simulink library "cylPackParChnlsLumped"  (R2025a)
settings: Solver=VariableStepAuto  StartTime=0.0  StopTime=10.0  RelTol=1e-3
undefined symbols (not defined in the file or in its folder): battery_builder_rtmsupport, gcbh
libraries: cylPackParChnlsLumped_lib x10, nesl_utility x3, batt_lib x1
(part 1 of 2)
settings Model: Creator=SimuVerity Contributors  LastModifiedBy=SimuVerity Contributors

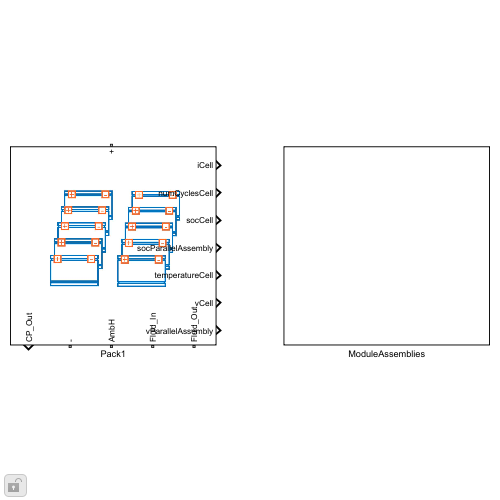
[thumbnail: Simulink's stored preview of the top-level diagram]
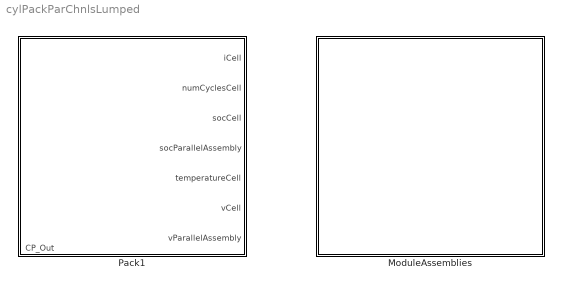
== system cylPackParChnlsLumped ==
  ModuleAssemblies : Subsystem
  Pack1 : Subsystem  LoadFcn=battery_builder_rtmsupport('loadfcn',gcbh);
      settings: CopyFcn=battery_builder_rtmsupport('copyfcn',gcbh);  PreCopyFcn=battery_builder_rtmsupport('precopyfcn',gcbh);  PreDeleteFcn=battery_builder_rtmsupport('predeletefcn',gcbh);  PortSchema="{\"entries\":[{\"content\":{\"sides\":[{\"content\":{\"connectorIds\":[\"LConn1\"]},\"type\":\"ConnectorPlacement.EquallySpacedRectSide\",\"uuid\":\"4681bb03-cd80-4246-89ba-52cf50faf921\"},{\"content\":{\"connectorIds\":[\"Out1\",\"RConn1\",\"RConn2\",\"RConn3\",\"RConn4\"],\"side\":\"RIGHT\"},\"type\":\"ConnectorPlacement.EquallySpacedRectSide\",\"uuid\":\"284cb137-d0f2-4bd0-b852-eba4066dd0c4\"},{\"content\":{\"side\":\"TOP\"},\"type\":\"ConnectorPlacement.EquallySpacedRectSide\",\"uuid\":\"dd50f81c-cf45-4e78-b3f5-c98c381b47a3\"},{\"content\":{\"connectorIds\":[\"Out2\",\"Out3\",\"Out4\",\"Out5\",\"Out6\",\"Out7\",\"Out8\"],\"side\":\"BOTTOM\"},\"type\":\"ConnectorPlacement.EquallySpacedRectSide\",\"uuid\":\"d30ee6a7-df81-42fc-8647-81cdeceb78f0\"}]},\"type\":\"ConnectorPlacement.EquallySpacedConnector\",\"uuid\":\"ee24a402-9efb-4b9e-88eb-dd7a5584ec7d\"}],\"packageUris\":[\"http://schema.mathworks.com/mf0/Connector/R2020b\"],\"version\":\"1.0\"}"
      mask Display: image('$imagefile')

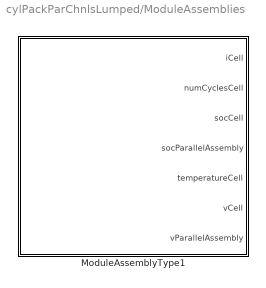
== system cylPackParChnlsLumped/ModuleAssemblies ==
  ModuleAssemblyType1 : Subsystem  LoadFcn=battery_builder_rtmsupport('loadfcn',gcbh);
      settings: CopyFcn=battery_builder_rtmsupport('copyfcn',gcbh);  PreCopyFcn=battery_builder_rtmsupport('precopyfcn',gcbh);  PreDeleteFcn=battery_builder_rtmsupport('predeletefcn',gcbh);  PortSchema="{\"entries\":[{\"content\":{\"sides\":[{\"content\":{\"connectorIds\":[\"LConn1\"]},\"type\":\"ConnectorPlacement.EquallySpacedRectSide\",\"uuid\":\"9f5d6674-91e5-41ab-bf84-a47b2d600243\"},{\"content\":{\"connectorIds\":[\"RConn1\",\"RConn2\",\"RConn3\"],\"side\":\"RIGHT\"},\"type\":\"ConnectorPlacement.EquallySpacedRectSide\",\"uuid\":\"fcae5f38-dd9a-4f90-b910-c15464afb2bd\"},{\"content\":{\"side\":\"TOP\"},\"type\":\"ConnectorPlacement.EquallySpacedRectSide\",\"uuid\":\"4b5634d1-8304-4a4e-97d4-9f8ecfb1b379\"},{\"content\":{\"connectorIds\":[\"Out1\",\"Out2\",\"Out3\",\"Out4\",\"Out5\",\"Out6\",\"Out7\"],\"side\":\"BOTTOM\"},\"type\":\"ConnectorPlacement.EquallySpacedRectSide\",\"uuid\":\"9ef905cb-dcbb-447b-9a1a-de2399b1e889\"}]},\"type\":\"ConnectorPlacement.EquallySpacedConnector\",\"uuid\":\"4a8d5c07-7366-4205-9241-e1a572108c18\"}],\"packageUris\":[\"http://schema.mathworks.com/mf0/Connector/R2020b\"],\"version\":\"1.0\"}"
      mask Display: image('$imagefile')

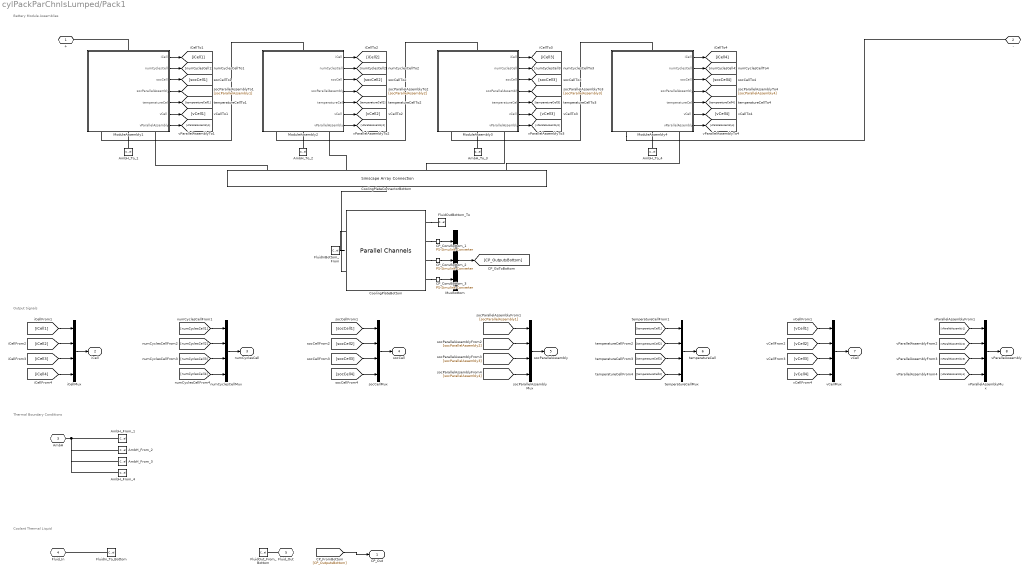
== system cylPackParChnlsLumped/Pack1 ==
  note: Battery Module Assemblies
  note: Output Signals
  note: Thermal Boundary Conditions
  note: Coolant Thermal Liquid
  AmbH_From_1 : ConnectionLabel  Label=ambH_1
  AmbH_From_2 : ConnectionLabel  Label=ambH_2
  AmbH_From_3 : ConnectionLabel  Label=ambH_3
  AmbH_From_4 : ConnectionLabel  Label=ambH_4
  AmbH_To_1 : ConnectionLabel  Label=ambH_1
  AmbH_To_2 : ConnectionLabel  Label=ambH_2
  AmbH_To_3 : ConnectionLabel  Label=ambH_3
  AmbH_To_4 : ConnectionLabel  Label=ambH_4
  CP_ConvBottom_1 : nesl_utility/PS-Simulink Converter  PhysicalDomain=network_engine_domain  SubClassName=ps_output  LeftPortType=input  RightPortType=output  PseudoPeriodic=off  Frequencies=[]  VectorFormat=inherit  Unit=inherit  AffineConversion=off
  CP_ConvBottom_2 : nesl_utility/PS-Simulink Converter  PhysicalDomain=network_engine_domain  SubClassName=ps_output  LeftPortType=input  RightPortType=output  PseudoPeriodic=off  Frequencies=[]  VectorFormat=inherit  Unit=inherit  AffineConversion=off
  CP_ConvBottom_3 : nesl_utility/PS-Simulink Converter  PhysicalDomain=network_engine_domain  SubClassName=ps_output  LeftPortType=input  RightPortType=output  PseudoPeriodic=off  Frequencies=[]  VectorFormat=inherit  Unit=inherit  AffineConversion=off
  CoolingPlateBottom : batt_lib/Thermal/Parallel Channels  plateConnectivity=simscape.battery.enum.thermal.coolingPlateConnectivity.singleSided  numBattThermalNodes1=CoolingPlateBottom.numBattThermalNodes1  dimensionThermalNodes1=CoolingPlateBottom.dimensionThermalNodes1  locationThermalNodes1=CoolingPlateBottom.locationThermalNodes1  numBattThermalNodes2=1  dimensionThermalNodes2=ones(1, 2)  locationThermalNodes2=ones(1, 2)  plateDimX=CoolingPlateBottom.plateDimX  plateDimY=CoolingPlateBottom.plateDimY  plateTh=CoolingPlateBottom.plateTh m  plateThCond=CoolingPlateBottom.plateThCond W/(K*m)  plateDen=CoolingPlateBottom.plateDen kg/m^3  plateCp=CoolingPlateBottom.plateCp J/(K*kg)  plateTemp_ini=CoolingPlateBottom.plateTemp_ini K  Re_lam=CoolingPlateBottom.Re_lam  Re_tur=CoolingPlateBottom.Re_tur  Nu_lam=CoolingPlateBottom.Nu_lam  length_add=CoolingPlateBottom.length_add m  shape_factor=CoolingPlateBottom.shape_factor  nChannels=CoolingPlateBottom.nChannels  selectChannelOrientation=simscape.battery.enum.thermal.coolingChannelsDirection.alongX  channelDia=CoolingPlateBottom.channelDia m  distributorDia=CoolingPlateBottom.distributorDia m  roughnessPipe=CoolingPlateBottom.roughnessPipe m
      settings: InternalSimscapePortConfiguration="{\"Bottom\":[],\"Left\":[{\"id\":\"fluid_in\",\"label\":\"fluid_in\",\"type\":\"foundation.thermal_liquid.thermal_liquid\"}],\"Right\":[{\"id\":\"fluid_out\",\"label\":\"fluid_out\",\"type\":\"foundation.thermal_liquid.thermal_liquid\"},{\"id\":\"plotPlateT\",\"label\":\"Tp\",\"type\":\"output\"},{\"id\":\"tempSensor\",\"label\":\"dT\",\"type\":\"output\"},{\"id\":\"presSensor\",\"label\":\"dP\",\"type\":\"output\"}],\"Top\":[{\"id\":\"Side1\",\"label\":\"Surf1\",\"type\":\"foundation.thermal.thermal\"}]}"
  CoolingPlateConnectorBottom : SimscapeArrayConnection  Domain=foundation.thermal.thermal  Mode=Sized Elements
  FluidInBottom_From : ConnectionLabel  Label=FluidIn_To_Bottom
  FluidIn_To_Bottom : ConnectionLabel  Label=FluidIn_To_Bottom
  FluidOutBottom_To : ConnectionLabel  Label=FluidOut_From_Bottom
  FluidOut_From_Bottom : ConnectionLabel  Label=FluidOut_From_Bottom
  ModuleAssembly1 : Subsystem  LoadFcn=battery_builder_rtmsupport('loadfcn',gcbh);
      settings: CopyFcn=battery_builder_rtmsupport('copyfcn',gcbh);  PreCopyFcn=battery_builder_rtmsupport('precopyfcn',gcbh);  PreDeleteFcn=battery_builder_rtmsupport('predeletefcn',gcbh);  PortSchema="{\"entries\":[{\"content\":{\"sides\":[{\"content\":{\"connectorIds\":[\"LConn1\"]},\"type\":\"ConnectorPlacement.EquallySpacedRectSide\",\"uuid\":\"9f5d6674-91e5-41ab-bf84-a47b2d600243\"},{\"content\":{\"connectorIds\":[\"RConn1\",\"RConn2\",\"RConn3\"],\"side\":\"RIGHT\"},\"type\":\"ConnectorPlacement.EquallySpacedRectSide\",\"uuid\":\"fcae5f38-dd9a-4f90-b910-c15464afb2bd\"},{\"content\":{\"side\":\"TOP\"},\"type\":\"ConnectorPlacement.EquallySpacedRectSide\",\"uuid\":\"4b5634d1-8304-4a4e-97d4-9f8ecfb1b379\"},{\"content\":{\"connectorIds\":[\"Out1\",\"Out2\",\"Out3\",\"Out4\",\"Out5\",\"Out6\",\"Out7\"],\"side\":\"BOTTOM\"},\"type\":\"ConnectorPlacement.EquallySpacedRectSide\",\"uuid\":\"9ef905cb-dcbb-447b-9a1a-de2399b1e889\"}]},\"type\":\"ConnectorPlacement.EquallySpacedConnector\",\"uuid\":\"4a8d5c07-7366-4205-9241-e1a572108c18\"}],\"packageUris\":[\"http://schema.mathworks.com/mf0/Connector/R2020b\"],\"version\":\"1.0\"}"
      mask Display: image('$imagefile')
  ModuleAssembly2 : Subsystem  LoadFcn=battery_builder_rtmsupport('loadfcn',gcbh);
      settings: CopyFcn=battery_builder_rtmsupport('copyfcn',gcbh);  PreCopyFcn=battery_builder_rtmsupport('precopyfcn',gcbh);  PreDeleteFcn=battery_builder_rtmsupport('predeletefcn',gcbh);  PortSchema="{\"entries\":[{\"content\":{\"sides\":[{\"content\":{\"connectorIds\":[\"LConn1\"]},\"type\":\"ConnectorPlacement.EquallySpacedRectSide\",\"uuid\":\"9f5d6674-91e5-41ab-bf84-a47b2d600243\"},{\"content\":{\"connectorIds\":[\"RConn1\",\"RConn2\",\"RConn3\"],\"side\":\"RIGHT\"},\"type\":\"ConnectorPlacement.EquallySpacedRectSide\",\"uuid\":\"fcae5f38-dd9a-4f90-b910-c15464afb2bd\"},{\"content\":{\"side\":\"TOP\"},\"type\":\"ConnectorPlacement.EquallySpacedRectSide\",\"uuid\":\"4b5634d1-8304-4a4e-97d4-9f8ecfb1b379\"},{\"content\":{\"connectorIds\":[\"Out1\",\"Out2\",\"Out3\",\"Out4\",\"Out5\",\"Out6\",\"Out7\"],\"side\":\"BOTTOM\"},\"type\":\"ConnectorPlacement.EquallySpacedRectSide\",\"uuid\":\"9ef905cb-dcbb-447b-9a1a-de2399b1e889\"}]},\"type\":\"ConnectorPlacement.EquallySpacedConnector\",\"uuid\":\"4a8d5c07-7366-4205-9241-e1a572108c18\"}],\"packageUris\":[\"http://schema.mathworks.com/mf0/Connector/R2020b\"],\"version\":\"1.0\"}"
      mask Display: image('$imagefile')
  ModuleAssembly3 : Subsystem  LoadFcn=battery_builder_rtmsupport('loadfcn',gcbh);
      settings: CopyFcn=battery_builder_rtmsupport('copyfcn',gcbh);  PreCopyFcn=battery_builder_rtmsupport('precopyfcn',gcbh);  PreDeleteFcn=battery_builder_rtmsupport('predeletefcn',gcbh);  PortSchema="{\"entries\":[{\"content\":{\"sides\":[{\"content\":{\"connectorIds\":[\"LConn1\"]},\"type\":\"ConnectorPlacement.EquallySpacedRectSide\",\"uuid\":\"9f5d6674-91e5-41ab-bf84-a47b2d600243\"},{\"content\":{\"connectorIds\":[\"RConn1\",\"RConn2\",\"RConn3\"],\"side\":\"RIGHT\"},\"type\":\"ConnectorPlacement.EquallySpacedRectSide\",\"uuid\":\"fcae5f38-dd9a-4f90-b910-c15464afb2bd\"},{\"content\":{\"side\":\"TOP\"},\"type\":\"ConnectorPlacement.EquallySpacedRectSide\",\"uuid\":\"4b5634d1-8304-4a4e-97d4-9f8ecfb1b379\"},{\"content\":{\"connectorIds\":[\"Out1\",\"Out2\",\"Out3\",\"Out4\",\"Out5\",\"Out6\",\"Out7\"],\"side\":\"BOTTOM\"},\"type\":\"ConnectorPlacement.EquallySpacedRectSide\",\"uuid\":\"9ef905cb-dcbb-447b-9a1a-de2399b1e889\"}]},\"type\":\"ConnectorPlacement.EquallySpacedConnector\",\"uuid\":\"4a8d5c07-7366-4205-9241-e1a572108c18\"}],\"packageUris\":[\"http://schema.mathworks.com/mf0/Connector/R2020b\"],\"version\":\"1.0\"}"
      mask Display: image('$imagefile')
  ModuleAssembly4 : Subsystem  LoadFcn=battery_builder_rtmsupport('loadfcn',gcbh);
      settings: CopyFcn=battery_builder_rtmsupport('copyfcn',gcbh);  PreCopyFcn=battery_builder_rtmsupport('precopyfcn',gcbh);  PreDeleteFcn=battery_builder_rtmsupport('predeletefcn',gcbh);  PortSchema="{\"entries\":[{\"content\":{\"sides\":[{\"content\":{\"connectorIds\":[\"LConn1\"]},\"type\":\"ConnectorPlacement.EquallySpacedRectSide\",\"uuid\":\"9f5d6674-91e5-41ab-bf84-a47b2d600243\"},{\"content\":{\"connectorIds\":[\"RConn1\",\"RConn2\",\"RConn3\"],\"side\":\"RIGHT\"},\"type\":\"ConnectorPlacement.EquallySpacedRectSide\",\"uuid\":\"fcae5f38-dd9a-4f90-b910-c15464afb2bd\"},{\"content\":{\"side\":\"TOP\"},\"type\":\"ConnectorPlacement.EquallySpacedRectSide\",\"uuid\":\"4b5634d1-8304-4a4e-97d4-9f8ecfb1b379\"},{\"content\":{\"connectorIds\":[\"Out1\",\"Out2\",\"Out3\",\"Out4\",\"Out5\",\"Out6\",\"Out7\"],\"side\":\"BOTTOM\"},\"type\":\"ConnectorPlacement.EquallySpacedRectSide\",\"uuid\":\"9ef905cb-dcbb-447b-9a1a-de2399b1e889\"}]},\"type\":\"ConnectorPlacement.EquallySpacedConnector\",\"uuid\":\"4a8d5c07-7366-4205-9241-e1a572108c18\"}],\"packageUris\":[\"http://schema.mathworks.com/mf0/Connector/R2020b\"],\"version\":\"1.0\"}"
      mask Display: image('$imagefile')
  MuxBottom : Mux  Inputs=3
  iCellMux : Mux
  numCyclesCellMux : Mux
  socCellMux : Mux
  socParallelAssemblyMux : Mux
  temperatureCellMux : Mux
  vCellMux : Mux
  vParallelAssemblyMux : Mux
  + : PMIOPort  Side=Left
  - : PMIOPort  Port=2  Side=Right
  AmbH : PMIOPort  Port=3  Side=Right  ConnectionType=Connection: foundation.thermal.thermal
  Fluid_In : PMIOPort  Port=4  Side=Right  ConnectionType=Connection: foundation.thermal_liquid.thermal_liquid
  Fluid_Out : PMIOPort  Port=5  Side=Right  ConnectionType=Connection: foundation.thermal_liquid.thermal_liquid
  CP_Out : Outport
  iCell : Outport  Port=2
  numCyclesCell : Outport  Port=3
  socCell : Outport  Port=4
  socParallelAssembly : Outport  Port=5
  temperatureCell : Outport  Port=6
  vCell : Outport  Port=7
  vParallelAssembly : Outport  Port=8
  wires:
  ModuleAssembly1/1(iCell) -> [iCell1]
  iCellMux/1 -> iCell/1
  [iCell1] -> iCellMux/1
  ModuleAssembly1/2(numCyclesCell) -> [numCyclesCell1]
  numCyclesCellMux/1 -> numCyclesCell/1
  [numCyclesCell1] -> numCyclesCellMux/1
  ModuleAssembly1/3(socCell) -> [socCell1]
  socCellMux/1 -> socCell/1
  [socCell1] -> socCellMux/1
  ModuleAssembly1/4(socParallelAssembly) -> [socParallelAssembly1]
  socParallelAssemblyMux/1 -> socParallelAssembly/1
  [socParallelAssembly1] -> socParallelAssemblyMux/1
  ModuleAssembly1/5(temperatureCell) -> [temperatureCell1]
  temperatureCellMux/1 -> temperatureCell/1
  [temperatureCell1] -> temperatureCellMux/1
  ModuleAssembly1/6(vCell) -> [vCell1]
  vCellMux/1 -> vCell/1
  [vCell1] -> vCellMux/1
  ModuleAssembly1/7(vParallelAssembly) -> [vParallelAssembly1]
  vParallelAssemblyMux/1 -> vParallelAssembly/1
  [vParallelAssembly1] -> vParallelAssemblyMux/1
  ModuleAssembly2/1(iCell) -> [iCell2]
  [iCell2] -> iCellMux/2
  ModuleAssembly2/2(numCyclesCell) -> [numCyclesCell2]
  [numCyclesCell2] -> numCyclesCellMux/2
  ModuleAssembly2/3(socCell) -> [socCell2]
  [socCell2] -> socCellMux/2
  ModuleAssembly2/4(socParallelAssembly) -> [socParallelAssembly2]
  [socParallelAssembly2] -> socParallelAssemblyMux/2
  ModuleAssembly2/5(temperatureCell) -> [temperatureCell2]
  [temperatureCell2] -> temperatureCellMux/2
  ModuleAssembly2/6(vCell) -> [vCell2]
  [vCell2] -> vCellMux/2
  ModuleAssembly2/7(vParallelAssembly) -> [vParallelAssembly2]
  [vParallelAssembly2] -> vParallelAssemblyMux/2
  ModuleAssembly3/1(iCell) -> [iCell3]
  [iCell3] -> iCellMux/3
  ModuleAssembly3/2(numCyclesCell) -> [numCyclesCell3]
  [numCyclesCell3] -> numCyclesCellMux/3
  ModuleAssembly3/3(socCell) -> [socCell3]
  [socCell3] -> socCellMux/3
  ModuleAssembly3/4(socParallelAssembly) -> [socParallelAssembly3]
  [socParallelAssembly3] -> socParallelAssemblyMux/3
  ModuleAssembly3/5(temperatureCell) -> [temperatureCell3]
  [temperatureCell3] -> temperatureCellMux/3
  ModuleAssembly3/6(vCell) -> [vCell3]
  [vCell3] -> vCellMux/3
  ModuleAssembly3/7(vParallelAssembly) -> [vParallelAssembly3]
  [vParallelAssembly3] -> vParallelAssemblyMux/3
  ModuleAssembly4/1(iCell) -> [iCell4]
  [iCell4] -> iCellMux/4
  ModuleAssembly4/2(numCyclesCell) -> [numCyclesCell4]
  [numCyclesCell4] -> numCyclesCellMux/4
  ModuleAssembly4/3(socCell) -> [socCell4]
  [socCell4] -> socCellMux/4
  ModuleAssembly4/4(socParallelAssembly) -> [socParallelAssembly4]
  [socParallelAssembly4] -> socParallelAssemblyMux/4
  ModuleAssembly4/5(temperatureCell) -> [temperatureCell4]
  [temperatureCell4] -> temperatureCellMux/4
  ModuleAssembly4/6(vCell) -> [vCell4]
  [vCell4] -> vCellMux/4
  ModuleAssembly4/7(vParallelAssembly) -> [vParallelAssembly4]
  [vParallelAssembly4] -> vParallelAssemblyMux/4
  CP_ConvBottom_1/1 -> MuxBottom/1
  CP_ConvBottom_2/1 -> MuxBottom/2
  CP_ConvBottom_3/1 -> MuxBottom/3
  MuxBottom/1 -> [CP_OutputsBottom]
  [CP_OutputsBottom] -> CP_Out/1
  connections:
  ModuleAssembly2/LConn1 -- ModuleAssembly1/RConn1
  ModuleAssembly3/LConn1 -- ModuleAssembly2/RConn1
  ModuleAssembly4/LConn1 -- ModuleAssembly3/RConn1
  ModuleAssembly1/LConn1 -- +/RConn1
  ModuleAssembly4/RConn1 -- -/RConn1
  AmbH_To_1/LConn1 -- ModuleAssembly1/RConn2
  AmbH_From_1/LConn1 -- AmbH_From_2/LConn1 -- AmbH_From_3/LConn1 -- AmbH/RConn1 -- AmbH_From_4/LConn1
  AmbH_To_2/LConn1 -- ModuleAssembly2/RConn2
  AmbH_To_3/LConn1 -- ModuleAssembly3/RConn2
  AmbH_To_4/LConn1 -- ModuleAssembly4/RConn2
  CoolingPlateConnectorBottom/LConn1 -- ModuleAssembly1/RConn3
  CoolingPlateConnectorBottom/LConn2 -- ModuleAssembly2/RConn3
  CoolingPlateConnectorBottom/LConn3 -- ModuleAssembly3/RConn3
  CoolingPlateConnectorBottom/LConn4 -- ModuleAssembly4/RConn3
  CoolingPlateConnectorBottom/RConn1 -- CoolingPlateBottom/LConn2
  FluidIn_To_Bottom/LConn1 -- Fluid_In/RConn1
  Fluid_Out/RConn1 -- FluidOut_From_Bottom/LConn1
  FluidInBottom_From/LConn1 -- CoolingPlateBottom/LConn1
  CoolingPlateBottom/RConn1 -- FluidOutBottom_To/LConn1
  CoolingPlateBottom/RConn2 -- CP_ConvBottom_1/LConn1
  CoolingPlateBottom/RConn3 -- CP_ConvBottom_2/LConn1
  CoolingPlateBottom/RConn4 -- CP_ConvBottom_3/LConn1

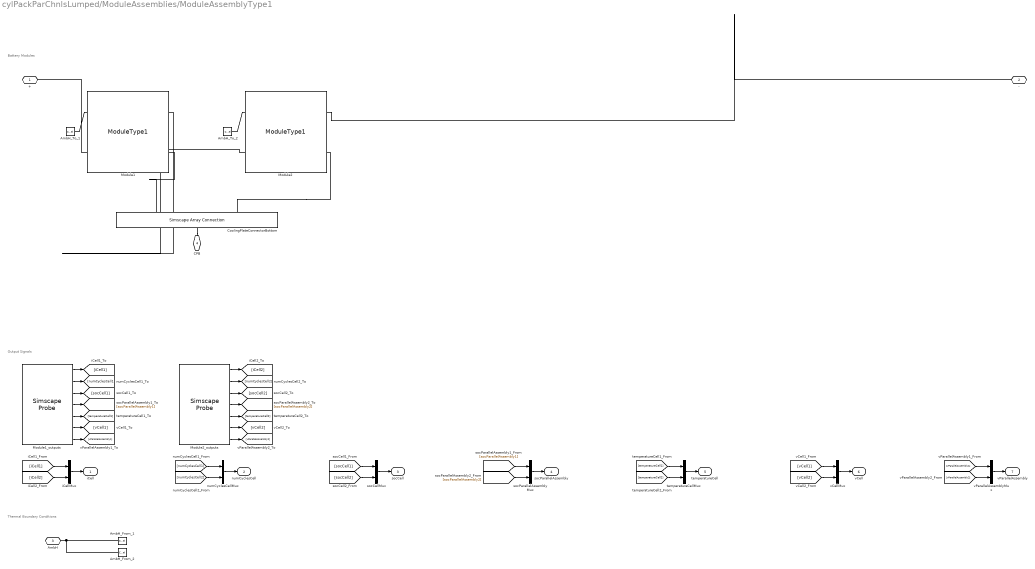
== system cylPackParChnlsLumped/ModuleAssemblies/ModuleAssemblyType1 ==
  note: Battery Modules
  note: Output Signals
  note: Thermal Boundary Conditions
  AmbH_From_1 : ConnectionLabel  Label=ambH_1
  AmbH_From_2 : ConnectionLabel  Label=ambH_2
  AmbH_To_1 : ConnectionLabel  Label=ambH_1
  AmbH_To_2 : ConnectionLabel  Label=ambH_2
  CoolingPlateConnectorBottom : SimscapeArrayConnection  Domain=foundation.thermal.thermal  Mode=Sized Elements
  Module1 : cylPackParChnlsLumped_lib/Modules/ModuleType1  SOC_vecCell=ModuleType1.SOC_vecCell  T_vecCell=ModuleType1.T_vecCell K  V0_matCell=ModuleType1.V0_matCell V  V_rangeCell=ModuleType1.V_rangeCell V  R0_matCell=ModuleType1.R0_matCell Ohm  AHCell=ModuleType1.AHCell A*hr  extrapolation_optionCell=simscape.enum.extrapolation.nearest  thermal_massCell=ModuleType1.thermal_massCell J/K  CoolantResistance=ModuleType1.CoolantResistance K/W  AmbientResistance=ModuleType1.AmbientResistance K/W  P=32  S=12  iCell_specify=off  iCell_priority=None  iCell=0 A  iCell_nominal_specify=off  iCell_nominal_value=1  iCell_nominal_unit=A  vCell_specify=off  vCell_priority=None  vCell=0 V  vCell_nominal_specify=off  vCell_nominal_value=1  vCell_nominal_unit=V  socCell_specify=off  socCell_priority=High  socCell=1  socCell_nominal_specify=off  socCell_nominal_value=1  socCell_nominal_unit=1  numCyclesCell_specify=off  numCyclesCell_priority=High  numCyclesCell=0  numCyclesCell_nominal_specify=off  numCyclesCell_nominal_value=1  numCyclesCell_nominal_unit=1  temperatureCell_specify=off  temperatureCell_priority=High  temperatureCell=298.15 K  temperatureCell_nominal_specify=off  temperatureCell_nominal_value=1  temperatureCell_nominal_unit=K  vParallelAssembly_specify=off  vParallelAssembly_priority=None  vParallelAssembly=repmat(0, 12, 1) V  vParallelAssembly_nominal_specify=off  vParallelAssembly_nominal_value=1  vParallelAssembly_nominal_unit=V  socParallelAssembly_specify=off  socParallelAssembly_priority=None  socParallelAssembly=repmat(1, 12, 1)  socParallelAssembly_nominal_specify=off  socParallelAssembly_nominal_value=1  socParallelAssembly_nominal_unit=1
      settings: InternalSimscapePortConfiguration="{\"Bottom\":[{\"id\":\"n\",\"label\":\"-\",\"type\":\"foundation.electrical.electrical\"},{\"id\":\"BottomExtClnt\",\"label\":\"CPB\",\"type\":\"foundation.thermal.thermal\"}],\"Left\":[{\"id\":\"AmbH\",\"label\":\"AmbH\",\"type\":\"foundation.thermal.thermal\"}],\"Right\":[],\"Top\":[{\"id\":\"p\",\"label\":\"+\",\"type\":\"foundation.electrical.electrical\"}]}"
  Module1_outputs : SimscapeProbe  BoundBlock=3  Variables="{\"iCell\":{\"Probing\":\"ON\"},\"numCyclesCell\":{\"Probing\":\"ON\"},\"socCell\":{\"Probing\":\"ON\"},\"socParallelAssembly\":{\"Probing\":\"ON\"},\"temperatureCell\":{\"Probing\":\"ON\"},\"vCell\":{\"Probing\":\"ON\"},\"vParallelAssembly\":{\"Probing\":\"ON\"}}"
  Module2 : cylPackParChnlsLumped_lib/Modules/ModuleType1  SOC_vecCell=ModuleType1.SOC_vecCell  T_vecCell=ModuleType1.T_vecCell K  V0_matCell=ModuleType1.V0_matCell V  V_rangeCell=ModuleType1.V_rangeCell V  R0_matCell=ModuleType1.R0_matCell Ohm  AHCell=ModuleType1.AHCell A*hr  extrapolation_optionCell=simscape.enum.extrapolation.nearest  thermal_massCell=ModuleType1.thermal_massCell J/K  CoolantResistance=ModuleType1.CoolantResistance K/W  AmbientResistance=ModuleType1.AmbientResistance K/W  P=32  S=12  iCell_specify=off  iCell_priority=None  iCell=0 A  iCell_nominal_specify=off  iCell_nominal_value=1  iCell_nominal_unit=A  vCell_specify=off  vCell_priority=None  vCell=0 V  vCell_nominal_specify=off  vCell_nominal_value=1  vCell_nominal_unit=V  socCell_specify=off  socCell_priority=High  socCell=1  socCell_nominal_specify=off  socCell_nominal_value=1  socCell_nominal_unit=1  numCyclesCell_specify=off  numCyclesCell_priority=High  numCyclesCell=0  numCyclesCell_nominal_specify=off  numCyclesCell_nominal_value=1  numCyclesCell_nominal_unit=1  temperatureCell_specify=off  temperatureCell_priority=High  temperatureCell=298.15 K  temperatureCell_nominal_specify=off  temperatureCell_nominal_value=1  temperatureCell_nominal_unit=K  vParallelAssembly_specify=off  vParallelAssembly_priority=None  vParallelAssembly=repmat(0, 12, 1) V  vParallelAssembly_nominal_specify=off  vParallelAssembly_nominal_value=1  vParallelAssembly_nominal_unit=V  socParallelAssembly_specify=off  socParallelAssembly_priority=None  socParallelAssembly=repmat(1, 12, 1)  socParallelAssembly_nominal_specify=off  socParallelAssembly_nominal_value=1  socParallelAssembly_nominal_unit=1
      settings: InternalSimscapePortConfiguration="{\"Bottom\":[{\"id\":\"n\",\"label\":\"-\",\"type\":\"foundation.electrical.electrical\"},{\"id\":\"BottomExtClnt\",\"label\":\"CPB\",\"type\":\"foundation.thermal.thermal\"}],\"Left\":[{\"id\":\"AmbH\",\"label\":\"AmbH\",\"type\":\"foundation.thermal.thermal\"}],\"Right\":[],\"Top\":[{\"id\":\"p\",\"label\":\"+\",\"type\":\"foundation.electrical.electrical\"}]}"
  Module2_outputs : SimscapeProbe  BoundBlock=4  Variables="{\"iCell\":{\"Probing\":\"ON\"},\"numCyclesCell\":{\"Probing\":\"ON\"},\"socCell\":{\"Probing\":\"ON\"},\"socParallelAssembly\":{\"Probing\":\"ON\"},\"temperatureCell\":{\"Probing\":\"ON\"},\"vCell\":{\"Probing\":\"ON\"},\"vParallelAssembly\":{\"Probing\":\"ON\"}}"
  iCellMux : Mux  Inputs=2
  numCyclesCellMux : Mux  Inputs=2
  socCellMux : Mux  Inputs=2
  socParallelAssemblyMux : Mux  Inputs=2
  temperatureCellMux : Mux  Inputs=2
  vCellMux : Mux  Inputs=2
  vParallelAssemblyMux : Mux  Inputs=2
  + : PMIOPort  Side=Left
  - : PMIOPort  Port=2  Side=Right
  AmbH : PMIOPort  Port=3  Side=Right  ConnectionType=Connection: foundation.thermal.thermal
  CPB : PMIOPort  Port=4  Side=Right  ConnectionType=Connection: foundation.thermal.thermal
  iCell : Outport
  numCyclesCell : Outport  Port=2
  socCell : Outport  Port=3
  socParallelAssembly : Outport  Port=4
  temperatureCell : Outport  Port=5
  vCell : Outport  Port=6
  vParallelAssembly : Outport  Port=7
  wires:
  Module1_outputs/1 -> [iCell1]
  iCellMux/1 -> iCell/1
  [iCell1] -> iCellMux/1
  Module1_outputs/2 -> [numCyclesCell1]
  numCyclesCellMux/1 -> numCyclesCell/1
  [numCyclesCell1] -> numCyclesCellMux/1
  Module1_outputs/3 -> [socCell1]
  socCellMux/1 -> socCell/1
  [socCell1] -> socCellMux/1
  Module1_outputs/4 -> [socParallelAssembly1]
  socParallelAssemblyMux/1 -> socParallelAssembly/1
  [socParallelAssembly1] -> socParallelAssemblyMux/1
  Module1_outputs/5 -> [temperatureCell1]
  temperatureCellMux/1 -> temperatureCell/1
  [temperatureCell1] -> temperatureCellMux/1
  Module1_outputs/6 -> [vCell1]
  vCellMux/1 -> vCell/1
  [vCell1] -> vCellMux/1
  Module1_outputs/7 -> [vParallelAssembly1]
  vParallelAssemblyMux/1 -> vParallelAssembly/1
  [vParallelAssembly1] -> vParallelAssemblyMux/1
  Module2_outputs/1 -> [iCell2]
  [iCell2] -> iCellMux/2
  Module2_outputs/2 -> [numCyclesCell2]
  [numCyclesCell2] -> numCyclesCellMux/2
  Module2_outputs/3 -> [socCell2]
  [socCell2] -> socCellMux/2
  Module2_outputs/4 -> [socParallelAssembly2]
  [socParallelAssembly2] -> socParallelAssemblyMux/2
  Module2_outputs/5 -> [temperatureCell2]
  [temperatureCell2] -> temperatureCellMux/2
  Module2_outputs/6 -> [vCell2]
  [vCell2] -> vCellMux/2
  Module2_outputs/7 -> [vParallelAssembly2]
  [vParallelAssembly2] -> vParallelAssemblyMux/2
  connections:
  Module2/LConn2 -- Module1/RConn1
  Module1/LConn2 -- +/RConn1
  Module2/RConn1 -- -/RConn1
  AmbH_To_1/LConn1 -- Module1/LConn1
  AmbH/RConn1 -- AmbH_From_1/LConn1 -- AmbH_From_2/LConn1
  AmbH_To_2/LConn1 -- Module2/LConn1
  CoolingPlateConnectorBottom/LConn1 -- Module1/RConn2
  CoolingPlateConnectorBottom/LConn2 -- Module2/RConn2
  CoolingPlateConnectorBottom/RConn1 -- CPB/RConn1

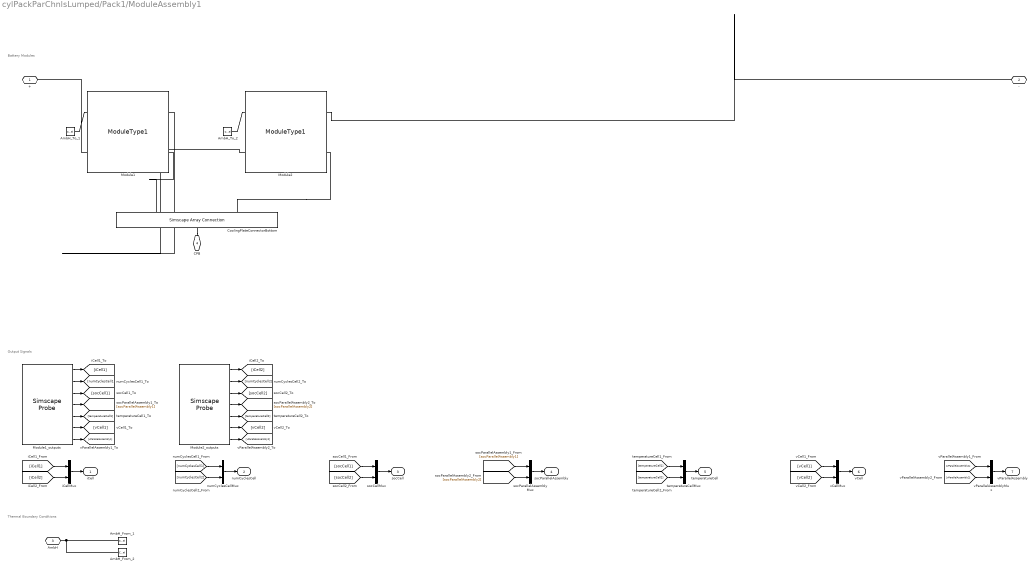
== system cylPackParChnlsLumped/Pack1/ModuleAssembly1 ==
  note: Thermal Boundary Conditions
  note: Output Signals
  note: Battery Modules
  AmbH_From_1 : ConnectionLabel  Label=ambH_1
  AmbH_From_2 : ConnectionLabel  Label=ambH_2
  AmbH_To_1 : ConnectionLabel  Label=ambH_1
  AmbH_To_2 : ConnectionLabel  Label=ambH_2
  CoolingPlateConnectorBottom : SimscapeArrayConnection  Domain=foundation.thermal.thermal  Mode=Sized Elements
  Module1 : cylPackParChnlsLumped_lib/Modules/ModuleType1  SOC_vecCell=ModuleType1.SOC_vecCell  T_vecCell=ModuleType1.T_vecCell K  V0_matCell=ModuleType1.V0_matCell V  V_rangeCell=ModuleType1.V_rangeCell V  R0_matCell=ModuleType1.R0_matCell Ohm  AHCell=ModuleType1.AHCell A*hr  extrapolation_optionCell=simscape.enum.extrapolation.nearest  thermal_massCell=ModuleType1.thermal_massCell J/K  CoolantResistance=ModuleType1.CoolantResistance K/W  AmbientResistance=ModuleType1.AmbientResistance K/W  P=32  S=12  iCell_specify=on  iCell_priority=None  iCell=ModuleAssembly1.Module1.iCell A  iCell_nominal_specify=off  iCell_nominal_value=1  iCell_nominal_unit=A  vCell_specify=on  vCell_priority=None  vCell=ModuleAssembly1.Module1.vCell V  vCell_nominal_specify=off  vCell_nominal_value=1  vCell_nominal_unit=V  socCell_specify=on  socCell_priority=High  socCell=ModuleAssembly1.Module1.socCell  socCell_nominal_specify=off  socCell_nominal_value=1  socCell_nominal_unit=1  numCyclesCell_specify=on  numCyclesCell_priority=High  numCyclesCell=ModuleAssembly1.Module1.numCyclesCell  numCyclesCell_nominal_specify=off  numCyclesCell_nominal_value=1  numCyclesCell_nominal_unit=1  temperatureCell_specify=on  temperatureCell_priority=High  temperatureCell=ModuleAssembly1.Module1.temperatureCell K  temperatureCell_nominal_specify=off  temperatureCell_nominal_value=1  temperatureCell_nominal_unit=K  vParallelAssembly_specify=on  vParallelAssembly_priority=None  vParallelAssembly=ModuleAssembly1.Module1.vParallelAssembly V  vParallelAssembly_nominal_specify=off  vParallelAssembly_nominal_value=1  vParallelAssembly_nominal_unit=V  socParallelAssembly_specify=on  socParallelAssembly_priority=None  socParallelAssembly=ModuleAssembly1.Module1.socParallelAssembly  socParallelAssembly_nominal_specify=off  socParallelAssembly_nominal_value=1  socParallelAssembly_nominal_unit=1
      settings: InternalSimscapePortConfiguration="{\"Bottom\":[{\"id\":\"n\",\"label\":\"-\",\"type\":\"foundation.electrical.electrical\"},{\"id\":\"BottomExtClnt\",\"label\":\"CPB\",\"type\":\"foundation.thermal.thermal\"}],\"Left\":[{\"id\":\"AmbH\",\"label\":\"AmbH\",\"type\":\"foundation.thermal.thermal\"}],\"Right\":[],\"Top\":[{\"id\":\"p\",\"label\":\"+\",\"type\":\"foundation.electrical.electrical\"}]}"
  Module1_outputs : SimscapeProbe  BoundBlock=68  Variables="{\"iCell\":{\"Probing\":\"ON\"},\"numCyclesCell\":{\"Probing\":\"ON\"},\"socCell\":{\"Probing\":\"ON\"},\"socParallelAssembly\":{\"Probing\":\"ON\"},\"temperatureCell\":{\"Probing\":\"ON\"},\"vCell\":{\"Probing\":\"ON\"},\"vParallelAssembly\":{\"Probing\":\"ON\"}}"
  Module2 : cylPackParChnlsLumped_lib/Modules/ModuleType1  SOC_vecCell=ModuleType1.SOC_vecCell  T_vecCell=ModuleType1.T_vecCell K  V0_matCell=ModuleType1.V0_matCell V  V_rangeCell=ModuleType1.V_rangeCell V  R0_matCell=ModuleType1.R0_matCell Ohm  AHCell=ModuleType1.AHCell A*hr  extrapolation_optionCell=simscape.enum.extrapolation.nearest  thermal_massCell=ModuleType1.thermal_massCell J/K  CoolantResistance=ModuleType1.CoolantResistance K/W  AmbientResistance=ModuleType1.AmbientResistance K/W  P=32  S=12  iCell_specify=on  iCell_priority=None  iCell=ModuleAssembly1.Module2.iCell A  iCell_nominal_specify=off  iCell_nominal_value=1  iCell_nominal_unit=A  vCell_specify=on  vCell_priority=None  vCell=ModuleAssembly1.Module2.vCell V  vCell_nominal_specify=off  vCell_nominal_value=1  vCell_nominal_unit=V  socCell_specify=on  socCell_priority=High  socCell=ModuleAssembly1.Module2.socCell  socCell_nominal_specify=off  socCell_nominal_value=1  socCell_nominal_unit=1  numCyclesCell_specify=on  numCyclesCell_priority=High  numCyclesCell=ModuleAssembly1.Module2.numCyclesCell  numCyclesCell_nominal_specify=off  numCyclesCell_nominal_value=1  numCyclesCell_nominal_unit=1  temperatureCell_specify=on  temperatureCell_priority=High  temperatureCell=ModuleAssembly1.Module2.temperatureCell K  temperatureCell_nominal_specify=off  temperatureCell_nominal_value=1  temperatureCell_nominal_unit=K  vParallelAssembly_specify=on  vParallelAssembly_priority=None  vParallelAssembly=ModuleAssembly1.Module2.vParallelAssembly V  vParallelAssembly_nominal_specify=off  vParallelAssembly_nominal_value=1  vParallelAssembly_nominal_unit=V  socParallelAssembly_specify=on  socParallelAssembly_priority=None  socParallelAssembly=ModuleAssembly1.Module2.socParallelAssembly  socParallelAssembly_nominal_specify=off  socParallelAssembly_nominal_value=1  socParallelAssembly_nominal_unit=1
      settings: InternalSimscapePortConfiguration="{\"Bottom\":[{\"id\":\"n\",\"label\":\"-\",\"type\":\"foundation.electrical.electrical\"},{\"id\":\"BottomExtClnt\",\"label\":\"CPB\",\"type\":\"foundation.thermal.thermal\"}],\"Left\":[{\"id\":\"AmbH\",\"label\":\"AmbH\",\"type\":\"foundation.thermal.thermal\"}],\"Right\":[],\"Top\":[{\"id\":\"p\",\"label\":\"+\",\"type\":\"foundation.electrical.electrical\"}]}"
  Module2_outputs : SimscapeProbe  BoundBlock=70  Variables="{\"iCell\":{\"Probing\":\"ON\"},\"numCyclesCell\":{\"Probing\":\"ON\"},\"socCell\":{\"Probing\":\"ON\"},\"socParallelAssembly\":{\"Probing\":\"ON\"},\"temperatureCell\":{\"Probing\":\"ON\"},\"vCell\":{\"Probing\":\"ON\"},\"vParallelAssembly\":{\"Probing\":\"ON\"}}"
  iCellMux : Mux  Inputs=2
  numCyclesCellMux : Mux  Inputs=2
  socCellMux : Mux  Inputs=2
  socParallelAssemblyMux : Mux  Inputs=2
  temperatureCellMux : Mux  Inputs=2
  vCellMux : Mux  Inputs=2
  vParallelAssemblyMux : Mux  Inputs=2
  + : PMIOPort  Side=Left
  - : PMIOPort  Port=2  Side=Right
  AmbH : PMIOPort  Port=3  Side=Right  ConnectionType=Connection: foundation.thermal.thermal
  CPB : PMIOPort  Port=4  Side=Right  ConnectionType=Connection: foundation.thermal.thermal
  iCell : Outport
  numCyclesCell : Outport  Port=2
  socCell : Outport  Port=3
  socParallelAssembly : Outport  Port=4
  temperatureCell : Outport  Port=5
  vCell : Outport  Port=6
  vParallelAssembly : Outport  Port=7
  wires:
  [vParallelAssembly2] -> vParallelAssemblyMux/2
  Module2_outputs/7 -> [vParallelAssembly2]
  [vCell2] -> vCellMux/2
  Module2_outputs/6 -> [vCell2]
  [temperatureCell2] -> temperatureCellMux/2
  Module2_outputs/5 -> [temperatureCell2]
  [socParallelAssembly2] -> socParallelAssemblyMux/2
  Module2_outputs/4 -> [socParallelAssembly2]
  [socCell2] -> socCellMux/2
  Module2_outputs/3 -> [socCell2]
  [numCyclesCell2] -> numCyclesCellMux/2
  Module2_outputs/2 -> [numCyclesCell2]
  [iCell2] -> iCellMux/2
  Module2_outputs/1 -> [iCell2]
  [vParallelAssembly1] -> vParallelAssemblyMux/1
  vParallelAssemblyMux/1 -> vParallelAssembly/1
  Module1_outputs/7 -> [vParallelAssembly1]
  [vCell1] -> vCellMux/1
  vCellMux/1 -> vCell/1
  Module1_outputs/6 -> [vCell1]
  [temperatureCell1] -> temperatureCellMux/1
  temperatureCellMux/1 -> temperatureCell/1
  Module1_outputs/5 -> [temperatureCell1]
  [socParallelAssembly1] -> socParallelAssemblyMux/1
  socParallelAssemblyMux/1 -> socParallelAssembly/1
  Module1_outputs/4 -> [socParallelAssembly1]
  [socCell1] -> socCellMux/1
  socCellMux/1 -> socCell/1
  Module1_outputs/3 -> [socCell1]
  [numCyclesCell1] -> numCyclesCellMux/1
  numCyclesCellMux/1 -> numCyclesCell/1
  Module1_outputs/2 -> [numCyclesCell1]
  [iCell1] -> iCellMux/1
  iCellMux/1 -> iCell/1
  Module1_outputs/1 -> [iCell1]
  connections:
  CoolingPlateConnectorBottom/RConn1 -- CPB/RConn1
  CoolingPlateConnectorBottom/LConn2 -- Module2/RConn2
  CoolingPlateConnectorBottom/LConn1 -- Module1/RConn2
  AmbH_To_2/LConn1 -- Module2/LConn1
  AmbH_From_2/LConn1 -- AmbH_From_1/LConn1 -- AmbH/RConn1
  AmbH_To_1/LConn1 -- Module1/LConn1
  Module2/RConn1 -- -/RConn1
  Module1/LConn2 -- +/RConn1
  Module2/LConn2 -- Module1/RConn1

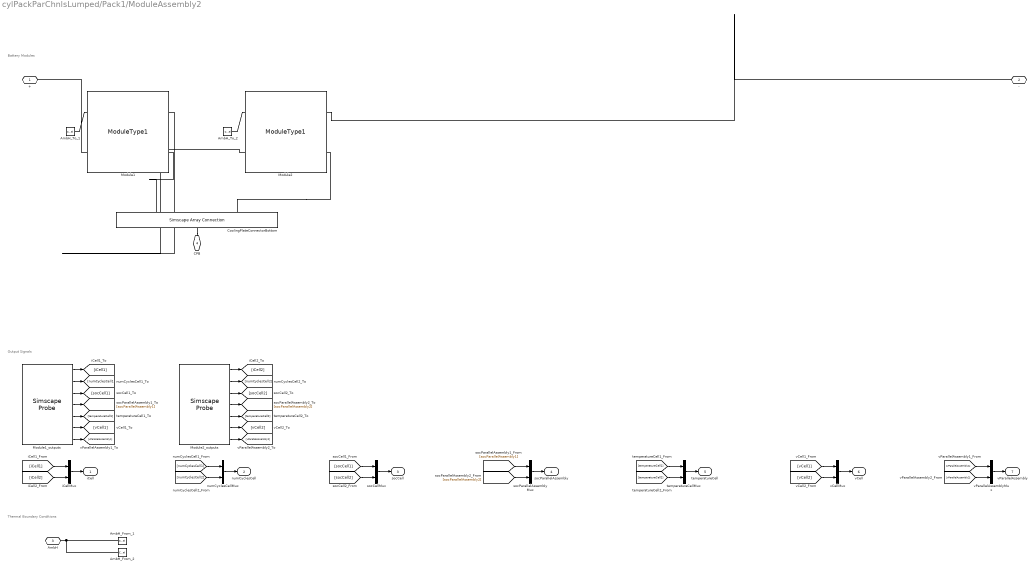
== system cylPackParChnlsLumped/Pack1/ModuleAssembly2 ==
  note: Thermal Boundary Conditions
  note: Output Signals
  note: Battery Modules
  AmbH_From_1 : ConnectionLabel  Label=ambH_1
  AmbH_From_2 : ConnectionLabel  Label=ambH_2
  AmbH_To_1 : ConnectionLabel  Label=ambH_1
  AmbH_To_2 : ConnectionLabel  Label=ambH_2
  CoolingPlateConnectorBottom : SimscapeArrayConnection  Domain=foundation.thermal.thermal  Mode=Sized Elements
  Module1 : cylPackParChnlsLumped_lib/Modules/ModuleType1  SOC_vecCell=ModuleType1.SOC_vecCell  T_vecCell=ModuleType1.T_vecCell K  V0_matCell=ModuleType1.V0_matCell V  V_rangeCell=ModuleType1.V_rangeCell V  R0_matCell=ModuleType1.R0_matCell Ohm  AHCell=ModuleType1.AHCell A*hr  extrapolation_optionCell=simscape.enum.extrapolation.nearest  thermal_massCell=ModuleType1.thermal_massCell J/K  CoolantResistance=ModuleType1.CoolantResistance K/W  AmbientResistance=ModuleType1.AmbientResistance K/W  P=32  S=12  iCell_specify=on  iCell_priority=None  iCell=ModuleAssembly2.Module1.iCell A  iCell_nominal_specify=off  iCell_nominal_value=1  iCell_nominal_unit=A  vCell_specify=on  vCell_priority=None  vCell=ModuleAssembly2.Module1.vCell V  vCell_nominal_specify=off  vCell_nominal_value=1  vCell_nominal_unit=V  socCell_specify=on  socCell_priority=High  socCell=ModuleAssembly2.Module1.socCell  socCell_nominal_specify=off  socCell_nominal_value=1  socCell_nominal_unit=1  numCyclesCell_specify=on  numCyclesCell_priority=High  numCyclesCell=ModuleAssembly2.Module1.numCyclesCell  numCyclesCell_nominal_specify=off  numCyclesCell_nominal_value=1  numCyclesCell_nominal_unit=1  temperatureCell_specify=on  temperatureCell_priority=High  temperatureCell=ModuleAssembly2.Module1.temperatureCell K  temperatureCell_nominal_specify=off  temperatureCell_nominal_value=1  temperatureCell_nominal_unit=K  vParallelAssembly_specify=on  vParallelAssembly_priority=None  vParallelAssembly=ModuleAssembly2.Module1.vParallelAssembly V  vParallelAssembly_nominal_specify=off  vParallelAssembly_nominal_value=1  vParallelAssembly_nominal_unit=V  socParallelAssembly_specify=on  socParallelAssembly_priority=None  socParallelAssembly=ModuleAssembly2.Module1.socParallelAssembly  socParallelAssembly_nominal_specify=off  socParallelAssembly_nominal_value=1  socParallelAssembly_nominal_unit=1
      settings: InternalSimscapePortConfiguration="{\"Bottom\":[{\"id\":\"n\",\"label\":\"-\",\"type\":\"foundation.electrical.electrical\"},{\"id\":\"BottomExtClnt\",\"label\":\"CPB\",\"type\":\"foundation.thermal.thermal\"}],\"Left\":[{\"id\":\"AmbH\",\"label\":\"AmbH\",\"type\":\"foundation.thermal.thermal\"}],\"Right\":[],\"Top\":[{\"id\":\"p\",\"label\":\"+\",\"type\":\"foundation.electrical.electrical\"}]}"
  Module1_outputs : SimscapeProbe  BoundBlock=127  Variables="{\"iCell\":{\"Probing\":\"ON\"},\"numCyclesCell\":{\"Probing\":\"ON\"},\"socCell\":{\"Probing\":\"ON\"},\"socParallelAssembly\":{\"Probing\":\"ON\"},\"temperatureCell\":{\"Probing\":\"ON\"},\"vCell\":{\"Probing\":\"ON\"},\"vParallelAssembly\":{\"Probing\":\"ON\"}}"
  Module2 : cylPackParChnlsLumped_lib/Modules/ModuleType1  SOC_vecCell=ModuleType1.SOC_vecCell  T_vecCell=ModuleType1.T_vecCell K  V0_matCell=ModuleType1.V0_matCell V  V_rangeCell=ModuleType1.V_rangeCell V  R0_matCell=ModuleType1.R0_matCell Ohm  AHCell=ModuleType1.AHCell A*hr  extrapolation_optionCell=simscape.enum.extrapolation.nearest  thermal_massCell=ModuleType1.thermal_massCell J/K  CoolantResistance=ModuleType1.CoolantResistance K/W  AmbientResistance=ModuleType1.AmbientResistance K/W  P=32  S=12  iCell_specify=on  iCell_priority=None  iCell=ModuleAssembly2.Module2.iCell A  iCell_nominal_specify=off  iCell_nominal_value=1  iCell_nominal_unit=A  vCell_specify=on  vCell_priority=None  vCell=ModuleAssembly2.Module2.vCell V  vCell_nominal_specify=off  vCell_nominal_value=1  vCell_nominal_unit=V  socCell_specify=on  socCell_priority=High  socCell=ModuleAssembly2.Module2.socCell  socCell_nominal_specify=off  socCell_nominal_value=1  socCell_nominal_unit=1  numCyclesCell_specify=on  numCyclesCell_priority=High  numCyclesCell=ModuleAssembly2.Module2.numCyclesCell  numCyclesCell_nominal_specify=off  numCyclesCell_nominal_value=1  numCyclesCell_nominal_unit=1  temperatureCell_specify=on  temperatureCell_priority=High  temperatureCell=ModuleAssembly2.Module2.temperatureCell K  temperatureCell_nominal_specify=off  temperatureCell_nominal_value=1  temperatureCell_nominal_unit=K  vParallelAssembly_specify=on  vParallelAssembly_priority=None  vParallelAssembly=ModuleAssembly2.Module2.vParallelAssembly V  vParallelAssembly_nominal_specify=off  vParallelAssembly_nominal_value=1  vParallelAssembly_nominal_unit=V  socParallelAssembly_specify=on  socParallelAssembly_priority=None  socParallelAssembly=ModuleAssembly2.Module2.socParallelAssembly  socParallelAssembly_nominal_specify=off  socParallelAssembly_nominal_value=1  socParallelAssembly_nominal_unit=1
      settings: InternalSimscapePortConfiguration="{\"Bottom\":[{\"id\":\"n\",\"label\":\"-\",\"type\":\"foundation.electrical.electrical\"},{\"id\":\"BottomExtClnt\",\"label\":\"CPB\",\"type\":\"foundation.thermal.thermal\"}],\"Left\":[{\"id\":\"AmbH\",\"label\":\"AmbH\",\"type\":\"foundation.thermal.thermal\"}],\"Right\":[],\"Top\":[{\"id\":\"p\",\"label\":\"+\",\"type\":\"foundation.electrical.electrical\"}]}"
  Module2_outputs : SimscapeProbe  BoundBlock=129  Variables="{\"iCell\":{\"Probing\":\"ON\"},\"numCyclesCell\":{\"Probing\":\"ON\"},\"socCell\":{\"Probing\":\"ON\"},\"socParallelAssembly\":{\"Probing\":\"ON\"},\"temperatureCell\":{\"Probing\":\"ON\"},\"vCell\":{\"Probing\":\"ON\"},\"vParallelAssembly\":{\"Probing\":\"ON\"}}"
  iCellMux : Mux  Inputs=2
  numCyclesCellMux : Mux  Inputs=2
  socCellMux : Mux  Inputs=2
  socParallelAssemblyMux : Mux  Inputs=2
  temperatureCellMux : Mux  Inputs=2
  vCellMux : Mux  Inputs=2
  vParallelAssemblyMux : Mux  Inputs=2
  + : PMIOPort  Side=Left
  - : PMIOPort  Port=2  Side=Right
  AmbH : PMIOPort  Port=3  Side=Right  ConnectionType=Connection: foundation.thermal.thermal
  CPB : PMIOPort  Port=4  Side=Right  ConnectionType=Connection: foundation.thermal.thermal
  iCell : Outport
  numCyclesCell : Outport  Port=2
  socCell : Outport  Port=3
  socParallelAssembly : Outport  Port=4
  temperatureCell : Outport  Port=5
  vCell : Outport  Port=6
  vParallelAssembly : Outport  Port=7
  wires:
  [vParallelAssembly2] -> vParallelAssemblyMux/2
  Module2_outputs/7 -> [vParallelAssembly2]
  [vCell2] -> vCellMux/2
  Module2_outputs/6 -> [vCell2]
  [temperatureCell2] -> temperatureCellMux/2
  Module2_outputs/5 -> [temperatureCell2]
  [socParallelAssembly2] -> socParallelAssemblyMux/2
  Module2_outputs/4 -> [socParallelAssembly2]
  [socCell2] -> socCellMux/2
  Module2_outputs/3 -> [socCell2]
  [numCyclesCell2] -> numCyclesCellMux/2
  Module2_outputs/2 -> [numCyclesCell2]
  [iCell2] -> iCellMux/2
  Module2_outputs/1 -> [iCell2]
  [vParallelAssembly1] -> vParallelAssemblyMux/1
  vParallelAssemblyMux/1 -> vParallelAssembly/1
  Module1_outputs/7 -> [vParallelAssembly1]
  [vCell1] -> vCellMux/1
  vCellMux/1 -> vCell/1
  Module1_outputs/6 -> [vCell1]
  [temperatureCell1] -> temperatureCellMux/1
  temperatureCellMux/1 -> temperatureCell/1
  Module1_outputs/5 -> [temperatureCell1]
  [socParallelAssembly1] -> socParallelAssemblyMux/1
  socParallelAssemblyMux/1 -> socParallelAssembly/1
  Module1_outputs/4 -> [socParallelAssembly1]
  [socCell1] -> socCellMux/1
  socCellMux/1 -> socCell/1
  Module1_outputs/3 -> [socCell1]
  [numCyclesCell1] -> numCyclesCellMux/1
  numCyclesCellMux/1 -> numCyclesCell/1
  Module1_outputs/2 -> [numCyclesCell1]
  [iCell1] -> iCellMux/1
  iCellMux/1 -> iCell/1
  Module1_outputs/1 -> [iCell1]
  connections:
  CoolingPlateConnectorBottom/RConn1 -- CPB/RConn1
  CoolingPlateConnectorBottom/LConn2 -- Module2/RConn2
  CoolingPlateConnectorBottom/LConn1 -- Module1/RConn2
  AmbH_To_2/LConn1 -- Module2/LConn1
  AmbH_From_2/LConn1 -- AmbH_From_1/LConn1 -- AmbH/RConn1
  AmbH_To_1/LConn1 -- Module1/LConn1
  Module2/RConn1 -- -/RConn1
  Module1/LConn2 -- +/RConn1
  Module2/LConn2 -- Module1/RConn1

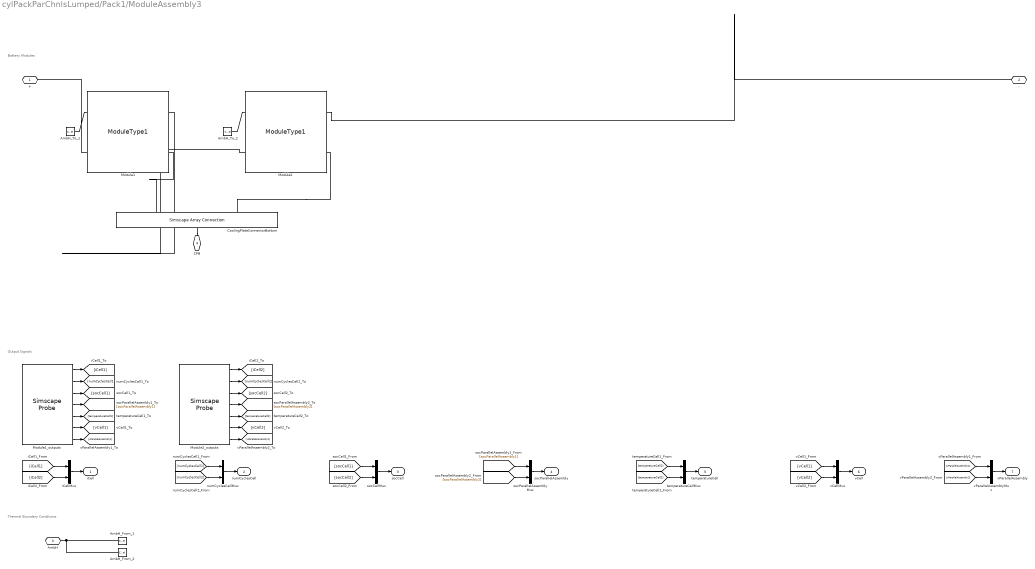
== system cylPackParChnlsLumped/Pack1/ModuleAssembly3 ==
  note: Thermal Boundary Conditions
  note: Output Signals
  note: Battery Modules
  AmbH_From_1 : ConnectionLabel  Label=ambH_1
  AmbH_From_2 : ConnectionLabel  Label=ambH_2
  AmbH_To_1 : ConnectionLabel  Label=ambH_1
  AmbH_To_2 : ConnectionLabel  Label=ambH_2
  CoolingPlateConnectorBottom : SimscapeArrayConnection  Domain=foundation.thermal.thermal  Mode=Sized Elements
  Module1 : cylPackParChnlsLumped_lib/Modules/ModuleType1  SOC_vecCell=ModuleType1.SOC_vecCell  T_vecCell=ModuleType1.T_vecCell K  V0_matCell=ModuleType1.V0_matCell V  V_rangeCell=ModuleType1.V_rangeCell V  R0_matCell=ModuleType1.R0_matCell Ohm  AHCell=ModuleType1.AHCell A*hr  extrapolation_optionCell=simscape.enum.extrapolation.nearest  thermal_massCell=ModuleType1.thermal_massCell J/K  CoolantResistance=ModuleType1.CoolantResistance K/W  AmbientResistance=ModuleType1.AmbientResistance K/W  P=32  S=12  iCell_specify=on  iCell_priority=None  iCell=ModuleAssembly3.Module1.iCell A  iCell_nominal_specify=off  iCell_nominal_value=1  iCell_nominal_unit=A  vCell_specify=on  vCell_priority=None  vCell=ModuleAssembly3.Module1.vCell V  vCell_nominal_specify=off  vCell_nominal_value=1  vCell_nominal_unit=V  socCell_specify=on  socCell_priority=High  socCell=ModuleAssembly3.Module1.socCell  socCell_nominal_specify=off  socCell_nominal_value=1  socCell_nominal_unit=1  numCyclesCell_specify=on  numCyclesCell_priority=High  numCyclesCell=ModuleAssembly3.Module1.numCyclesCell  numCyclesCell_nominal_specify=off  numCyclesCell_nominal_value=1  numCyclesCell_nominal_unit=1  temperatureCell_specify=on  temperatureCell_priority=High  temperatureCell=ModuleAssembly3.Module1.temperatureCell K  temperatureCell_nominal_specify=off  temperatureCell_nominal_value=1  temperatureCell_nominal_unit=K  vParallelAssembly_specify=on  vParallelAssembly_priority=None  vParallelAssembly=ModuleAssembly3.Module1.vParallelAssembly V  vParallelAssembly_nominal_specify=off  vParallelAssembly_nominal_value=1  vParallelAssembly_nominal_unit=V  socParallelAssembly_specify=on  socParallelAssembly_priority=None  socParallelAssembly=ModuleAssembly3.Module1.socParallelAssembly  socParallelAssembly_nominal_specify=off  socParallelAssembly_nominal_value=1  socParallelAssembly_nominal_unit=1
      settings: InternalSimscapePortConfiguration="{\"Bottom\":[{\"id\":\"n\",\"label\":\"-\",\"type\":\"foundation.electrical.electrical\"},{\"id\":\"BottomExtClnt\",\"label\":\"CPB\",\"type\":\"foundation.thermal.thermal\"}],\"Left\":[{\"id\":\"AmbH\",\"label\":\"AmbH\",\"type\":\"foundation.thermal.thermal\"}],\"Right\":[],\"Top\":[{\"id\":\"p\",\"label\":\"+\",\"type\":\"foundation.electrical.electrical\"}]}"
  Module1_outputs : SimscapeProbe  BoundBlock=186  Variables="{\"iCell\":{\"Probing\":\"ON\"},\"numCyclesCell\":{\"Probing\":\"ON\"},\"socCell\":{\"Probing\":\"ON\"},\"socParallelAssembly\":{\"Probing\":\"ON\"},\"temperatureCell\":{\"Probing\":\"ON\"},\"vCell\":{\"Probing\":\"ON\"},\"vParallelAssembly\":{\"Probing\":\"ON\"}}"
  Module2 : cylPackParChnlsLumped_lib/Modules/ModuleType1  SOC_vecCell=ModuleType1.SOC_vecCell  T_vecCell=ModuleType1.T_vecCell K  V0_matCell=ModuleType1.V0_matCell V  V_rangeCell=ModuleType1.V_rangeCell V  R0_matCell=ModuleType1.R0_matCell Ohm  AHCell=ModuleType1.AHCell A*hr  extrapolation_optionCell=simscape.enum.extrapolation.nearest  thermal_massCell=ModuleType1.thermal_massCell J/K  CoolantResistance=ModuleType1.CoolantResistance K/W  AmbientResistance=ModuleType1.AmbientResistance K/W  P=32  S=12  iCell_specify=on  iCell_priority=None  iCell=ModuleAssembly3.Module2.iCell A  iCell_nominal_specify=off  iCell_nominal_value=1  iCell_nominal_unit=A  vCell_specify=on  vCell_priority=None  vCell=ModuleAssembly3.Module2.vCell V  vCell_nominal_specify=off  vCell_nominal_value=1  vCell_nominal_unit=V  socCell_specify=on  socCell_priority=High  socCell=ModuleAssembly3.Module2.socCell  socCell_nominal_specify=off  socCell_nominal_value=1  socCell_nominal_unit=1  numCyclesCell_specify=on  numCyclesCell_priority=High  numCyclesCell=ModuleAssembly3.Module2.numCyclesCell  numCyclesCell_nominal_specify=off  numCyclesCell_nominal_value=1  numCyclesCell_nominal_unit=1  temperatureCell_specify=on  temperatureCell_priority=High  temperatureCell=ModuleAssembly3.Module2.temperatureCell K  temperatureCell_nominal_specify=off  temperatureCell_nominal_value=1  temperatureCell_nominal_unit=K  vParallelAssembly_specify=on  vParallelAssembly_priority=None  vParallelAssembly=ModuleAssembly3.Module2.vParallelAssembly V  vParallelAssembly_nominal_specify=off  vParallelAssembly_nominal_value=1  vParallelAssembly_nominal_unit=V  socParallelAssembly_specify=on  socParallelAssembly_priority=None  socParallelAssembly=ModuleAssembly3.Module2.socParallelAssembly  socParallelAssembly_nominal_specify=off  socParallelAssembly_nominal_value=1  socParallelAssembly_nominal_unit=1
      settings: InternalSimscapePortConfiguration="{\"Bottom\":[{\"id\":\"n\",\"label\":\"-\",\"type\":\"foundation.electrical.electrical\"},{\"id\":\"BottomExtClnt\",\"label\":\"CPB\",\"type\":\"foundation.thermal.thermal\"}],\"Left\":[{\"id\":\"AmbH\",\"label\":\"AmbH\",\"type\":\"foundation.thermal.thermal\"}],\"Right\":[],\"Top\":[{\"id\":\"p\",\"label\":\"+\",\"type\":\"foundation.electrical.electrical\"}]}"
  Module2_outputs : SimscapeProbe  BoundBlock=188  Variables="{\"iCell\":{\"Probing\":\"ON\"},\"numCyclesCell\":{\"Probing\":\"ON\"},\"socCell\":{\"Probing\":\"ON\"},\"socParallelAssembly\":{\"Probing\":\"ON\"},\"temperatureCell\":{\"Probing\":\"ON\"},\"vCell\":{\"Probing\":\"ON\"},\"vParallelAssembly\":{\"Probing\":\"ON\"}}"
  iCellMux : Mux  Inputs=2
  numCyclesCellMux : Mux  Inputs=2
  socCellMux : Mux  Inputs=2
  socParallelAssemblyMux : Mux  Inputs=2
  temperatureCellMux : Mux  Inputs=2
  vCellMux : Mux  Inputs=2
  vParallelAssemblyMux : Mux  Inputs=2
  + : PMIOPort  Side=Left
  - : PMIOPort  Port=2  Side=Right
  AmbH : PMIOPort  Port=3  Side=Right  ConnectionType=Connection: foundation.thermal.thermal
  CPB : PMIOPort  Port=4  Side=Right  ConnectionType=Connection: foundation.thermal.thermal
  iCell : Outport
  numCyclesCell : Outport  Port=2
  socCell : Outport  Port=3
  socParallelAssembly : Outport  Port=4
  temperatureCell : Outport  Port=5
  vCell : Outport  Port=6
  vParallelAssembly : Outport  Port=7
  wires:
  [vParallelAssembly2] -> vParallelAssemblyMux/2
  Module2_outputs/7 -> [vParallelAssembly2]
  [vCell2] -> vCellMux/2
  Module2_outputs/6 -> [vCell2]
  [temperatureCell2] -> temperatureCellMux/2
  Module2_outputs/5 -> [temperatureCell2]
  [socParallelAssembly2] -> socParallelAssemblyMux/2
  Module2_outputs/4 -> [socParallelAssembly2]
  [socCell2] -> socCellMux/2
  Module2_outputs/3 -> [socCell2]
  [numCyclesCell2] -> numCyclesCellMux/2
  Module2_outputs/2 -> [numCyclesCell2]
  [iCell2] -> iCellMux/2
  Module2_outputs/1 -> [iCell2]
  [vParallelAssembly1] -> vParallelAssemblyMux/1
  vParallelAssemblyMux/1 -> vParallelAssembly/1
  Module1_outputs/7 -> [vParallelAssembly1]
  [vCell1] -> vCellMux/1
  vCellMux/1 -> vCell/1
  Module1_outputs/6 -> [vCell1]
  [temperatureCell1] -> temperatureCellMux/1
  temperatureCellMux/1 -> temperatureCell/1
  Module1_outputs/5 -> [temperatureCell1]
  [socParallelAssembly1] -> socParallelAssemblyMux/1
  socParallelAssemblyMux/1 -> socParallelAssembly/1
  Module1_outputs/4 -> [socParallelAssembly1]
  [socCell1] -> socCellMux/1
  socCellMux/1 -> socCell/1
  Module1_outputs/3 -> [socCell1]
  [numCyclesCell1] -> numCyclesCellMux/1
  numCyclesCellMux/1 -> numCyclesCell/1
  Module1_outputs/2 -> [numCyclesCell1]
  [iCell1] -> iCellMux/1
  iCellMux/1 -> iCell/1
  Module1_outputs/1 -> [iCell1]
  connections:
  CoolingPlateConnectorBottom/RConn1 -- CPB/RConn1
  CoolingPlateConnectorBottom/LConn2 -- Module2/RConn2
  CoolingPlateConnectorBottom/LConn1 -- Module1/RConn2
  AmbH_To_2/LConn1 -- Module2/LConn1
  AmbH_From_2/LConn1 -- AmbH_From_1/LConn1 -- AmbH/RConn1
  AmbH_To_1/LConn1 -- Module1/LConn1
  Module2/RConn1 -- -/RConn1
  Module1/LConn2 -- +/RConn1
  Module2/LConn2 -- Module1/RConn1
